simulink model "assignment3"  (R2026a)
settings: Solver=VariableStepAuto  StopTime=10^6  MaxStep=0.01
values from neighbouring files (symbols this model uses):
  A = 1    [assignment3_param.m]
  k = 10    [assignment3_param.m]
  omega = 100    [assignment3_param.m]
settings Model: Creator=saradenti  LastModifiedBy=saradenti

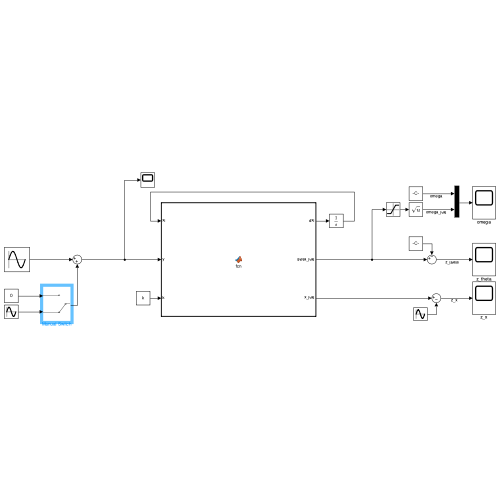
[thumbnail: Simulink's stored preview of the top-level diagram]
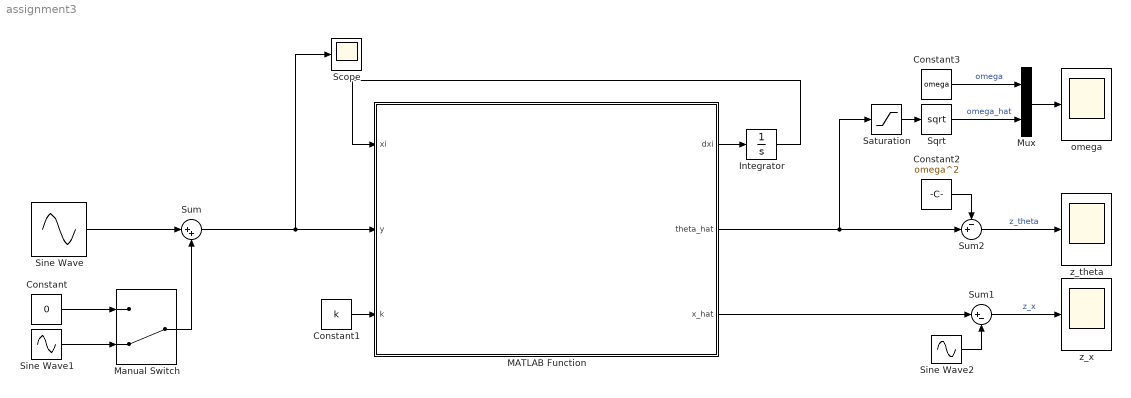
== system assignment3 ==
  Constant : Constant  Value=0
  Constant1 : Constant  Value=k
  Constant2 : Constant  Value=omega^2
  Constant3 : Constant  Value=omega
  Integrator : Integrator  InitialCondition=[0; 0]
  MATLAB Function : MATLAB Function  TreatAsAtomicUnit=on
  Manual Switch : ManualSwitch  CurrentSetting=0
  Mux : Mux  Inputs=2
  Saturation : Saturate  UpperLimit=inf  LowerLimit=0
  Scope : Scope
      settings: ActiveDisplayYMinimum=0.82149034347211658  ActiveDisplayYMaximum=1.0428255200937782  DataLoggingVariableName=ScopeData3
  Sine Wave : Sin  Amplitude=A  Frequency=omega  SampleTime=0
  Sine Wave1 : Sin  Amplitude=0.001  Frequency=50  SampleTime=0
  Sine Wave2 : Sin  Amplitude=A*omega  Frequency=omega  Phase=pi/2  SampleTime=0
  Sqrt : Sqrt
  Sum : Sum  Inputs=|++
  Sum1 : Sum  Inputs=|+-
  Sum2 : Sum  Inputs=-+|
  omega : Scope
      settings: ActiveDisplayYMinimum=99.995505341793887  ActiveDisplayYMaximum=100.00224656242084  DataLoggingVariableName=ScopeData2
  z_theta : Scope
      settings: ActiveDisplayYMinimum=-1  ActiveDisplayYMaximum=1
  z_x : Scope
      settings: ActiveDisplayYMinimum=-325.87391647752531  ActiveDisplayYMaximum=267.4650560675899
  wires:
  Sine Wave/1 -> Sum/1
  Manual Switch/1 -> Sum/2
  Constant/1 -> Manual Switch/1
  Sine Wave1/1 -> Manual Switch/2
  Sum/1 -> Scope/1, MATLAB Function/2(y)
  MATLAB Function/1(dxi) -> Integrator/1
  Integrator/1 -> MATLAB Function/1(xi)
  Constant1/1 -> MATLAB Function/3(k)
  Sum1/1 -> z_x/1  "z_x"
  Sum2/1 -> z_theta/1  "z_theta"
  MATLAB Function/3(x_hat) -> Sum1/1
  Sine Wave2/1 -> Sum1/2
  MATLAB Function/2(theta_hat) -> Saturation/1, Sum2/2
  Constant2/1 -> Sum2/1
  Mux/1 -> omega/1
  Constant3/1 -> Mux/1  "omega"
  Sqrt/1 -> Mux/2  "omega_hat"
  Saturation/1 -> Sqrt/1

== matlab function assignment3/MATLAB Function ==
  data: xi input; y input; k input; dxi output; theta_hat output; x_hat output
function [dxi, theta_hat,  x_hat] = fcn(xi, y, k)

    dxi = zeros(2,1);

    dxi(1) = - k * xi(1) - y;
    dxi(2) = - xi(1)^2 * (k^2 + xi(1) * y + xi(2)) + y^2;

    theta_hat = xi(1) * y + xi(2);
    x_hat = k * y + (k^2 + theta_hat) * xi(1);
